simulink subsystem "M8025_Actuator"  (R2025b)
settings: Solver=VariableStepAuto  StartTime=0.0  StopTime=10.0  RelTol=1e-3
model mask{VelKp=0.00076207895, VelKi=0.0015241579}
  mask prompts: VelKp "Velocity Kp"; VelKi "Velocity Ki"
undefined symbols (not defined in the file): M8025
libraries: fl_lib x12, nesl_utility x9, slpidlib x2, ee_lib x1
settings Model: Creator=Compu  LastModifiedBy=Compu

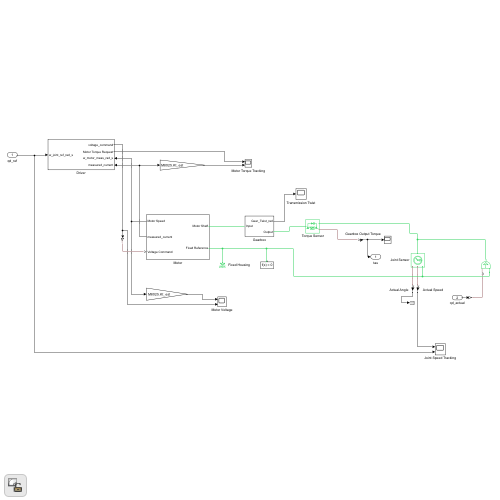
[thumbnail: Simulink's stored preview of the top-level diagram]
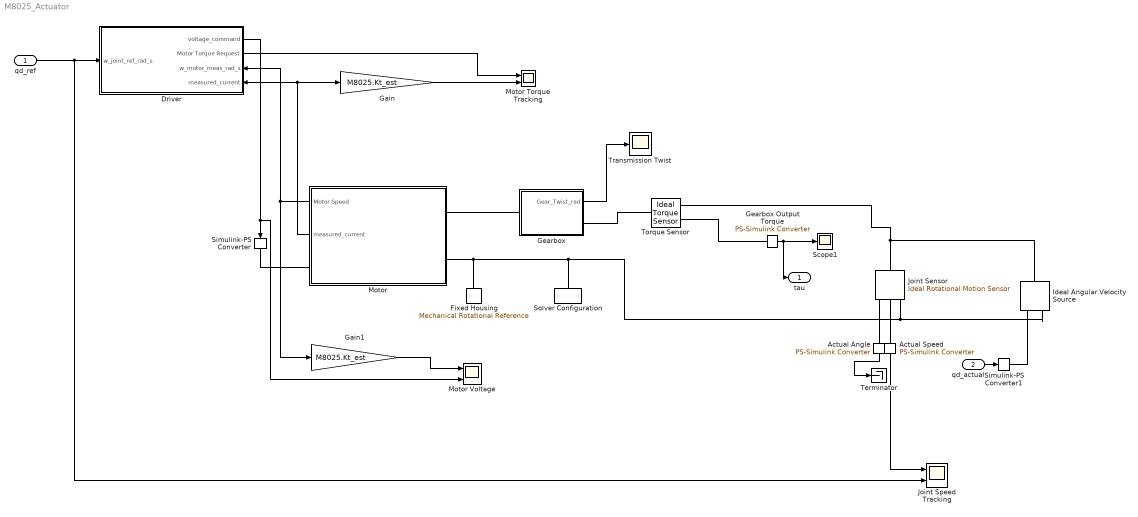
== system M8025_Actuator ==
  qd_ref : Inport
  qd_actual : Inport  Port=2
  Actual Angle : nesl_utility/PS-Simulink Converter  PhysicalDomain=network_engine_domain  SubClassName=ps_output  LeftPortType=input  RightPortType=output  PseudoPeriodic=off  Frequencies=[]  VectorFormat=inherit  Unit=rad  AffineConversion=off
  Actual Speed : nesl_utility/PS-Simulink Converter  PhysicalDomain=network_engine_domain  SubClassName=ps_output  LeftPortType=input  RightPortType=output  PseudoPeriodic=off  Frequencies=[]  VectorFormat=inherit  Unit=rad/s  AffineConversion=off
  Driver : Subsystem
      settings: PortSchema="{\"entries\":[{\"content\":{\"sides\":[{\"content\":{\"connectorIds\":[\"In1\"]},\"type\":\"ConnectorPlacement.EquallySpacedRectSide\",\"uuid\":\"4f9c6ada-d4f2-4042-b799-7a5129c92780\"},{\"content\":{\"connectorIds\":[\"Out1\",\"Out2\",\"In2\",\"In3\"],\"side\":\"RIGHT\"},\"type\":\"ConnectorPlacement.EquallySpacedRectSide\",\"uuid\":\"e7c5d0cc-560f-4bd8-9eed-f21f11202f3f\"},{\"content\":{\"side\":\"TOP\"},\"type\":\"ConnectorPlacement.EquallySpacedRectSide\",\"uuid\":\"9d50fcf4-e910-4695-a284-862e67cc701d\"}]},\"type\":\"ConnectorPlacement.EquallySpacedConnector\",\"uuid\":\"3eedfdac-378a-49e8-9696-691ddb81d7b7\"}],\"packageUris\":[\"http://schema.mathworks.com/mf0/Connector/R2020b\"],\"version\":\"1.0\"}"
  Fixed Housing : fl_lib/Mechanical/Rotational Elements/Mechanical Rotational Reference
  Gain : Gain  Gain=M8025.Kt_est
  Gain1 : Gain  Gain=M8025.Kt_est
  Gearbox : Subsystem
  Gearbox Output Torque : nesl_utility/PS-Simulink Converter  PhysicalDomain=network_engine_domain  SubClassName=ps_output  LeftPortType=input  RightPortType=output  PseudoPeriodic=off  Frequencies=[]  VectorFormat=inherit  Unit=N*m  AffineConversion=off
  Ideal Angular Velocity Source : fl_lib/Mechanical/Mechanical Sources/Ideal Angular Velocity Source
  Joint Sensor : fl_lib/Mechanical/Mechanical Sensors/Ideal Rotational Motion Sensor  reference=foundation.enum.MeasurementReference.difference  acceleration_port=false  velocity_port=true  position_port=true  wrap_angle=false  offset=0 rad
  Joint Speed Tracking : Scope  NumInputPorts=2
      settings: ActiveDisplayYMinimum=-0.02793  ActiveDisplayYMaximum=0.25141  DataLoggingVariableName=ScopeData2
  Motor : Subsystem
      settings: PortSchema="{\"entries\":[{\"content\":{\"sides\":[{\"content\":{\"connectorIds\":[\"Out1\",\"Out2\",\"LConn1\"]},\"type\":\"ConnectorPlacement.EquallySpacedRectSide\",\"uuid\":\"a7d9d3e7-63ba-44cc-8810-cbbe49fdc417\"},{\"content\":{\"connectorIds\":[\"RConn1\",\"RConn2\"],\"side\":\"RIGHT\"},\"type\":\"ConnectorPlacement.EquallySpacedRectSide\",\"uuid\":\"fa3b5d3d-db74-48e3-94ee-4f6883535878\"},{\"content\":{\"side\":\"TOP\"},\"type\":\"ConnectorPlacement.EquallySpacedRectSide\",\"uuid\":\"19ef0f19-9e47-4a9a-82bb-e035ff550378\"}]},\"type\":\"ConnectorPlacement.EquallySpacedConnector\",\"uuid\":\"8a6ad2f5-5551-4596-9ab7-1b2bcec8fe13\"}],\"packageUris\":[\"http://schema.mathworks.com/mf0/Connector/R2020b\"],\"version\":\"1.0\"}"
  Motor Torque Tracking : Scope  NumInputPorts=2
      settings: ActiveDisplayYMinimum=-0.00179  ActiveDisplayYMaximum=0.01392
  Motor Voltage : Scope  NumInputPorts=2
      settings: ActiveDisplayYMinimum=-0.49501  ActiveDisplayYMaximum=4.45509  DataLoggingVariableName=ScopeData4
  Scope1 : Scope
  Simulink-PS Converter : nesl_utility/Simulink-PS Converter  PhysicalDomain=network_engine_domain  SubClassName=ps_input  LeftPortType=input  RightPortType=output  PseudoPeriodic=off  Frequencies=[]  NoiseDistribution=none  NoiseParameters=[]  Unit=V  AffineConversion=off  FilteringAndDerivatives=provide  SimscapeFilterOrder=1  InputFilterTimeConstant=0.001  UdotUserProvided=0
  Simulink-PS Converter1 : nesl_utility/Simulink-PS Converter  PhysicalDomain=network_engine_domain  SubClassName=ps_input  LeftPortType=input  RightPortType=output  PseudoPeriodic=off  Frequencies=[]  NoiseDistribution=none  NoiseParameters=[]  Unit=1  AffineConversion=off  FilteringAndDerivatives=provide  SimscapeFilterOrder=1  InputFilterTimeConstant=0.001  UdotUserProvided=0
  Solver Configuration : nesl_utility/Solver Configuration  PhysicalDomain=network_engine_domain  SubClassName=solver  LeftPortType=input  RightPortType=generic  Tones=[]  Harmonics=[]  SimulateNoise=off  Profile=off  UseLocalSampling=off  EnableSwitchedLinearOptims=on  FrequencyDomain=off  UseCCode=off  RelTol=0.001  AbsTol=0.001  MinStep=1e-09  ToWorkspace=off  RevertToSquareIcSolve=off  NumHomotopyIterations=100  PhasorMode=off  PhasorModeNumHarmonics=1  ConsistencySolver=NEWTON_XTOL_AFTER_FTOL  IndexReductionMethod=DerivativeReplacement  DoDC=off  ResidualTolerance=1e-09  ConsistencyTolSource=GLOBAL  ConsistencyAbsTol=0.001  ConsistencyRelTol=0.001  ConsistencyTolFactor=0.001  UseLocalSolver=off  LocalSolverChoice=NE_BACKWARD_EULER_ADVANCER  ResolveIndetEquations=on  FunctionEvalNumThread=1  LocalSolverSampleTime=0.001  DoFixedCost=off  MaxNonlinIter=3  MaxModeIter=2  ComputeImpulses=off  ImpulseIterations=2  LinearAlgebra=auto  LinearAlgebraNumThread=0  EquationFormulation=NE_TIME_EF  DelaysMemoryBudget=1024  AutomaticFiltering=on  FilteringTimeConstant=0.001  PartitionStorageMethod=AS_NEEDED  PartitionMemoryBudget=1024  PartitionMethod=ROBUST  MultibodyUseLocalSolver=off  MultibodyLocalSolverChoice=ODE1  MultibodyLocalSolverSampleTime=0.001
  Terminator : Terminator
  Torque Sensor : fl_lib/Mechanical/Mechanical Sensors/Ideal Torque Sensor
  Transmission Twist : Scope
      settings: ActiveDisplayYMinimum=-2E-6  ActiveDisplayYMaximum=2E-5  DataLoggingVariableName=ScopeData5
  tau : Outport
  wires:
  Actual Speed/1 -> Joint Speed Tracking/1
  qd_actual/1 -> Simulink-PS Converter1/1
  Driver/1(voltage_command) -> Simulink-PS Converter/1, Motor Voltage/2
  qd_ref/1 -> Driver/1(w_joint_ref_rad_s), Joint Speed Tracking/2
  Motor/2(measured_current) -> Driver/3(measured_current), Gain/1
  Gearbox Output Torque/1 -> Scope1/1, tau/1
  Driver/2(Motor Torque Request) -> Motor Torque Tracking/1
  Actual Angle/1 -> Terminator/1
  Motor/1(Motor Speed) -> Driver/2(w_motor_meas_rad_s), Gain1/1
  Gain/1 -> Motor Torque Tracking/2
  Gain1/1 -> Motor Voltage/1
  Gearbox/1(Gear_Twist_rad) -> Transmission Twist/1
  connections:
  Fixed Housing/LConn1 -- Joint Sensor/RConn1 -- Ideal Angular Velocity Source/RConn2 -- Solver Configuration/RConn1 -- Motor/RConn2
  Ideal Angular Velocity Source/LConn1 -- Joint Sensor/LConn1 -- Torque Sensor/RConn1
  Torque Sensor/RConn2 -- Gearbox Output Torque/LConn1
  Simulink-PS Converter1/RConn1 -- Ideal Angular Velocity Source/RConn1
  Simulink-PS Converter/RConn1 -- Motor/LConn1
  Joint Sensor/RConn2 -- Actual Speed/LConn1
  Gearbox/RConn1 -- Torque Sensor/LConn1
  Motor/RConn1 -- Gearbox/LConn1
  Joint Sensor/RConn3 -- Actual Angle/LConn1

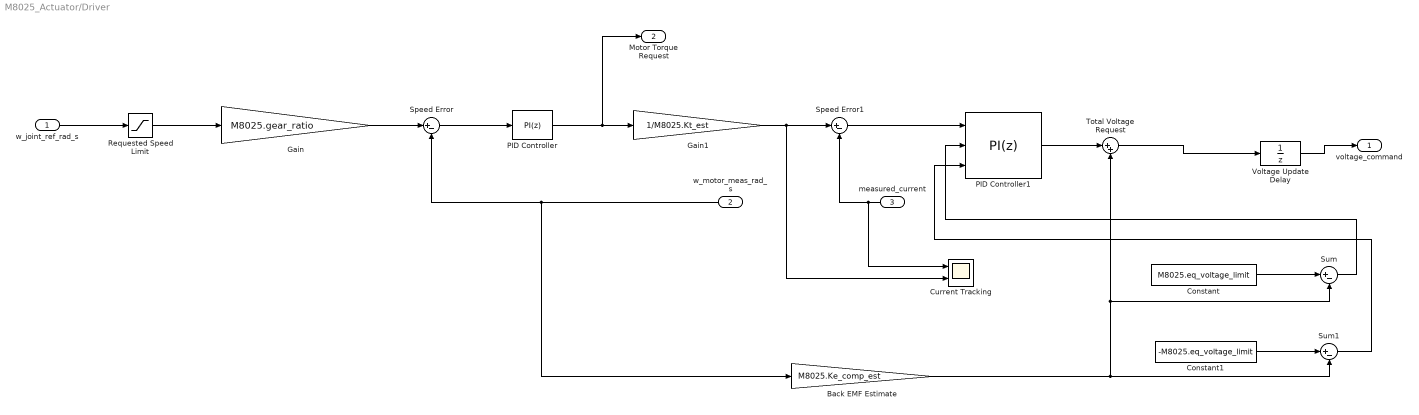
== system M8025_Actuator/Driver ==
  w_joint_ref_rad_s : Inport
  w_motor_meas_rad_s : Inport  Port=2
  measured_current : Inport  Port=3
  Back EMF Estimate : Gain  Gain=M8025.Ke_comp_est
  Constant : Constant  Value=M8025.eq_voltage_limit
  Constant1 : Constant  Value=-M8025.eq_voltage_limit
  Current Tracking : Scope  NumInputPorts=2
      settings: ActiveDisplayYMinimum=-0.00854  ActiveDisplayYMaximum=0.06628  DataLoggingVariableName=ScopeData3
  Gain : Gain  Gain=M8025.gear_ratio
  Gain1 : Gain  Gain=1/M8025.Kt_est
  PID Controller : slpidlib/PID Controller  Controller=PI  Form=Parallel  TimeDomain=Discrete-time  UseExternalTs=off  SampleTime=0.0001  IntegratorMethod=Forward Euler  FilterMethod=Forward Euler  ControllerParametersSource=internal  P=VelKp  I=VelKi  UseKiTs=off  D=0  UseExternalDerivativeSource=off  N=100  UseFilter=on  TunerSelectOption=Transfer Function Based (PID Tuner App)  InitialConditionSource=internal  InitialConditionForIntegrator=0  InitialConditionForFilter=0  DifferentiatorICPrevScaledInput=0  ExternalReset=none  TrackingMode=off  Kt=1  LimitOutput=on  SatLimitsSource=internal  UpperSaturationLimit=M8025.rated_output_torque/M8025.gear_ratio  LowerSaturationLimit=-M8025.rated_output_torque/M8025.gear_ratio  LinearizeAsGain=on  AntiWindupMode=clamping  Kb=1  LimitIntegrator=off  UpperIntegratorSaturationLimit=inf  LowerIntegratorSaturationLimit=-inf  POutMin=[]  POutMax=[]  IOutMin=[]  IOutMax=[]  DOutMin=[]  DOutMax=[]  NOutMin=[]  NOutMax=[]  SumOutMin=[]  SumOutMax=[]  SaturationOutMin=[]  SaturationOutMax=[]  PParamMin=[]  PParamMax=[]  IParamMin=[]  IParamMax=[]  DParamMin=[]  DParamMax=[]  NParamMin=[]  NParamMax=[]  KbParamMin=[]  KbParamMax=[]  KtParamMin=[]  KtParamMax=[]  KbOutMin=[]  KbOutMax=[]  KtOutMin=[]  KtOutMax=[]  IntegratorOutMin=[]  IntegratorOutMax=[]  FilterOutMin=[]  FilterOutMax=[]  SumI1OutMin=[]  SumI1OutMax=[]  SumI2OutMin=[]  SumI2OutMax=[]  SumI3OutMin=[]  SumI3OutMax=[]  SumI4OutMin=[]  SumI4OutMax=[]  SumDOutMin=[]  SumDOutMax=[]  DifferentiatorOutMin=[]  DifferentiatorOutMax=[]  FilterDiffOutCoefMin=[]  FilterDiffOutCoefMax=[]  ReciprocalOutMin=[]  ReciprocalOutMax=[]  SumDenOutMin=[]  SumDenOutMax=[]  SumNumOutMin=[]  SumNumOutMax=[]  DivideOutMin=[]  DivideOutMax=[]  UdiffTsProdOutMin=[]  UdiffTsProdOutMax=[]  NTsProdOutMin=[]  NTsProdOutMax=[]  UintegralTsProdOutMin=[]  UintegralTsProdOutMax=[]  UngainTsProdOutMin=[]  UngainTsProdOutMax=[]  ClampingZeroOutDataTypeStr=Inherit: Inherit via back propagation  ClampingZeroOutMin=[]  ClampingZeroOutMax=[]  FilterDenConstantOutDataTypeStr=Inherit: Inherit via back propagation  FilterDenConstantOutMin=[]  FilterDenConstantOutMax=[]  PCopyOutDataTypeStr=Inherit: Inherit via back propagation  PCopyOutMin=[]  PCopyOutMax=[]  NCopyOutDataTypeStr=Inherit: Inherit via back propagation  NCopyOutMin=[]  NCopyOutMax=[]  IntegratorContinuousStateAttributes=''  IntegratorStateMustResolveToSignalObject=off  IntegratorRTWStateStorageClass=Auto  FilterContinuousStateAttributes=''  FilterStateMustResolveToSignalObject=off  FilterRTWStateStorageClass=Auto  ParallelPVariant=InternalParameters  IdealPVariant=Disabled  IVariant=InternalParameters  DVariant=Disabled  IntegratorVariant=Discrete  SatVariant=Enabled  AWVariant=DiscClampingParallel  PCopyVariant=Disabled  TRVariant=Disabled  FdbkBlocksVariant=Forward  IdealPFdbkVariant=Disabled  SatFdbkVariant=Disabled  DerivativeFilterVariant=Disabled  NVariant=Disabled  NCopyVariant=Disabled_SignalSpec  FilterICVariant=Disabled  IntegratorICVariant=InternalICs  ExternalResetVariant=Disabled  TRSumVariant=Passthrough  SumFdbkVariant=Disabled  SumVariant=Sum_PI  TsampFilterVariant=InternalTs  TsampNgainVariant=Passthrough  TsampIntegralVariant=Disabled_SignalSpec  ExternalSaturationOutDataTypeStr=Inherit: Same as second input  DerivativeSourceVariant=Disabled  PreIntVariant=InternalPreInt
  PID Controller1 : slpidlib/PID Controller  Controller=PI  Form=Parallel  TimeDomain=Discrete-time  UseExternalTs=off  SampleTime=0.0001  IntegratorMethod=Forward Euler  FilterMethod=Forward Euler  ControllerParametersSource=internal  P=M8025.current_P_design  I=M8025.current_I_design  UseKiTs=off  D=0  UseExternalDerivativeSource=off  N=100  UseFilter=on  TunerSelectOption=Transfer Function Based (PID Tuner App)  InitialConditionSource=internal  InitialConditionForIntegrator=0  InitialConditionForFilter=0  DifferentiatorICPrevScaledInput=0  ExternalReset=none  TrackingMode=off  Kt=1  LimitOutput=on  SatLimitsSource=external  UpperSaturationLimit=M8025.eq_voltage_limit  LowerSaturationLimit=-M8025.eq_voltage_limit  LinearizeAsGain=on  AntiWindupMode=clamping  Kb=1  LimitIntegrator=off  UpperIntegratorSaturationLimit=inf  LowerIntegratorSaturationLimit=-inf  POutMin=[]  POutMax=[]  IOutMin=[]  IOutMax=[]  DOutMin=[]  DOutMax=[]  NOutMin=[]  NOutMax=[]  SumOutMin=[]  SumOutMax=[]  SaturationOutMin=[]  SaturationOutMax=[]  PParamMin=[]  PParamMax=[]  IParamMin=[]  IParamMax=[]  DParamMin=[]  DParamMax=[]  NParamMin=[]  NParamMax=[]  KbParamMin=[]  KbParamMax=[]  KtParamMin=[]  KtParamMax=[]  KbOutMin=[]  KbOutMax=[]  KtOutMin=[]  KtOutMax=[]  IntegratorOutMin=[]  IntegratorOutMax=[]  FilterOutMin=[]  FilterOutMax=[]  SumI1OutMin=[]  SumI1OutMax=[]  SumI2OutMin=[]  SumI2OutMax=[]  SumI3OutMin=[]  SumI3OutMax=[]  SumI4OutMin=[]  SumI4OutMax=[]  SumDOutMin=[]  SumDOutMax=[]  DifferentiatorOutMin=[]  DifferentiatorOutMax=[]  FilterDiffOutCoefMin=[]  FilterDiffOutCoefMax=[]  ReciprocalOutMin=[]  ReciprocalOutMax=[]  SumDenOutMin=[]  SumDenOutMax=[]  SumNumOutMin=[]  SumNumOutMax=[]  DivideOutMin=[]  DivideOutMax=[]  UdiffTsProdOutMin=[]  UdiffTsProdOutMax=[]  NTsProdOutMin=[]  NTsProdOutMax=[]  UintegralTsProdOutMin=[]  UintegralTsProdOutMax=[]  UngainTsProdOutMin=[]  UngainTsProdOutMax=[]  ClampingZeroOutDataTypeStr=Inherit: Inherit via back propagation  ClampingZeroOutMin=[]  ClampingZeroOutMax=[]  FilterDenConstantOutDataTypeStr=Inherit: Inherit via back propagation  FilterDenConstantOutMin=[]  FilterDenConstantOutMax=[]  PCopyOutDataTypeStr=Inherit: Inherit via back propagation  PCopyOutMin=[]  PCopyOutMax=[]  NCopyOutDataTypeStr=Inherit: Inherit via back propagation  NCopyOutMin=[]  NCopyOutMax=[]  IntegratorContinuousStateAttributes=''  IntegratorStateMustResolveToSignalObject=off  IntegratorRTWStateStorageClass=Auto  FilterContinuousStateAttributes=''  FilterStateMustResolveToSignalObject=off  FilterRTWStateStorageClass=Auto  ParallelPVariant=InternalParameters  IdealPVariant=Disabled  IVariant=InternalParameters  DVariant=Disabled  IntegratorVariant=Discrete  SatVariant=External  AWVariant=DiscClampingParallel  PCopyVariant=Disabled  TRVariant=Disabled  FdbkBlocksVariant=Forward  IdealPFdbkVariant=Disabled  SatFdbkVariant=Disabled  DerivativeFilterVariant=Disabled  NVariant=Disabled  NCopyVariant=Disabled_SignalSpec  FilterICVariant=Disabled  IntegratorICVariant=InternalICs  ExternalResetVariant=Disabled  TRSumVariant=Passthrough  SumFdbkVariant=Disabled  SumVariant=Sum_PI  TsampFilterVariant=InternalTs  TsampNgainVariant=Passthrough  TsampIntegralVariant=Disabled_SignalSpec  ExternalSaturationOutDataTypeStr=Inherit: Same as second input  DerivativeSourceVariant=Disabled  PreIntVariant=InternalPreInt
  Requested Speed Limit : Saturate  UpperLimit=1.885  LowerLimit=-1.885
  Speed Error : Sum  Inputs=|+-
  Speed Error1 : Sum  Inputs=|+-
  Sum : Sum  Inputs=|+-
  Sum1 : Sum  Inputs=|+-
  Total Voltage Request : Sum  Inputs=|++
  Voltage Update Delay : UnitDelay  SampleTime=0.0001  HasFrameUpgradeWarning=on
  voltage_command : Outport
  Motor Torque Request : Outport  Port=2
  wires:
  Constant1/1 -> Sum1/1
  Sum1/1 -> PID Controller1/3
  Sum/1 -> PID Controller1/2
  Constant/1 -> Sum/1
  PID Controller1/1 -> Total Voltage Request/1
  Back EMF Estimate/1 -> Sum/2, Total Voltage Request/2, Sum1/2
  measured_current/1 -> Speed Error1/2, Current Tracking/1
  Speed Error1/1 -> PID Controller1/1
  Gain1/1 -> Speed Error1/1, Current Tracking/2
  PID Controller/1 -> Gain1/1, Motor Torque Request/1
  w_joint_ref_rad_s/1 -> Requested Speed Limit/1
  Gain/1 -> Speed Error/1
  Speed Error/1 -> PID Controller/1
  Requested Speed Limit/1 -> Gain/1
  w_motor_meas_rad_s/1 -> Back EMF Estimate/1, Speed Error/2
  Total Voltage Request/1 -> Voltage Update Delay/1
  Voltage Update Delay/1 -> voltage_command/1

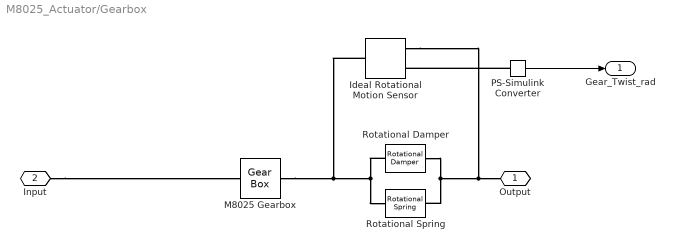
== system M8025_Actuator/Gearbox ==
  Ideal Rotational Motion Sensor : fl_lib/Mechanical/Mechanical Sensors/Ideal Rotational Motion Sensor  reference=foundation.enum.MeasurementReference.difference  acceleration_port=false  velocity_port=false  position_port=true  wrap_angle=false  offset=0 rad
      settings: InternalSimscapePortConfiguration="{\"Bottom\":[],\"Left\":[{\"id\":\"R\",\"label\":\"R\",\"type\":\"foundation.mechanical.rotational.rotational\"}],\"Right\":[{\"id\":\"C\",\"label\":\"C\",\"type\":\"foundation.mechanical.rotational.rotational\"},{\"id\":\"A\",\"label\":\"A\",\"type\":\"output\"}],\"Top\":[]}"
  M8025 Gearbox : fl_lib/Mechanical/Mechanisms/Gear Box  ratio=M8025.gear_ratio  t_in_specify=off  t_in_priority=None  t_in=0 N*m  t_in_nominal_specify=off  t_in_nominal_value=1  t_in_nominal_unit=N*m  t_out_specify=off  t_out_priority=None  t_out=0 N*m  t_out_nominal_specify=off  t_out_nominal_value=1  t_out_nominal_unit=N*m
  PS-Simulink Converter : nesl_utility/PS-Simulink Converter  PhysicalDomain=network_engine_domain  SubClassName=ps_output  LeftPortType=input  RightPortType=output  PseudoPeriodic=off  Frequencies=[]  VectorFormat=inherit  Unit=rad  AffineConversion=off
  Rotational Damper : fl_lib/Mechanical/Rotational Elements/Rotational Damper  D=M8025.gear_damping_trial N*m*s/rad  w_specify=off  w_priority=None  w=0 rad/s  w_nominal_specify=off  w_nominal_value=1  w_nominal_unit=rad/s  t_specify=off  t_priority=None  t=0 N*m  t_nominal_specify=off  t_nominal_value=1  t_nominal_unit=N*m
  Rotational Spring : fl_lib/Mechanical/Rotational Elements/Rotational Spring  spr_rate=M8025.gear_stiffness_trial N*m/rad  w_specify=off  w_priority=None  w=0 rad/s  w_nominal_specify=off  w_nominal_value=1  w_nominal_unit=rad/s  t_specify=off  t_priority=None  t=0 N*m  t_nominal_specify=off  t_nominal_value=1  t_nominal_unit=N*m  phi_specify=off  phi_priority=High  phi=0 rad  phi_nominal_specify=off  phi_nominal_value=1  phi_nominal_unit=rad
  Output : PMIOPort  Side=Right
  Input : PMIOPort  Port=2  Side=Left
  Gear_Twist_rad : Outport
  wires:
  PS-Simulink Converter/1 -> Gear_Twist_rad/1
  connections:
  PS-Simulink Converter/LConn1 -- Ideal Rotational Motion Sensor/RConn2
  Rotational Spring/RConn1 -- Output/RConn1 -- Ideal Rotational Motion Sensor/RConn1 -- Rotational Damper/RConn1
  Rotational Spring/LConn1 -- M8025 Gearbox/RConn1 -- Ideal Rotational Motion Sensor/LConn1 -- Rotational Damper/LConn1
  Input/RConn1 -- M8025 Gearbox/LConn1

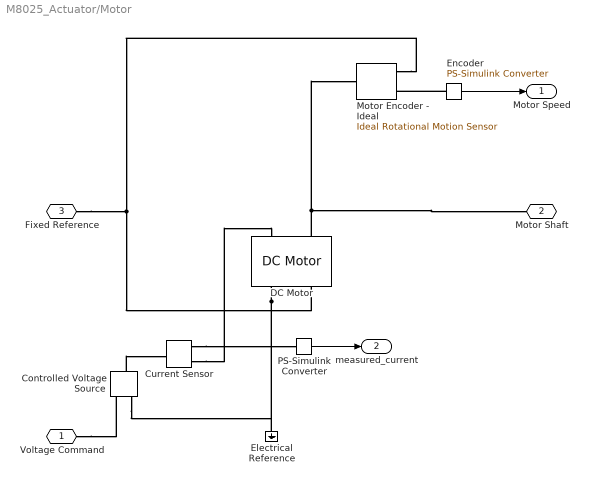
== system M8025_Actuator/Motor ==
  Controlled Voltage Source : fl_lib/Electrical/Electrical Sources/Controlled Voltage Source
  Current Sensor : fl_lib/Electrical/Electrical Sensors/Current Sensor
  DC Motor : ee_lib/Electromechanical/Brushed Motors/DC Motor  field_option=ee.enum.field_option.pm  Rf=100 Ohm  Lf=1 H  Laf=0.15 H  If0=0 A  parameterization=ee.enum.dcparam_option.circuit_param  Ra=M8025.eq_R Ohm  La=M8025.eq_L H  emf_or_torque=ee.enum.emf_or_torque.ki  Kv=0.072e-3 V/rpm  Ki=M8025.Kt_est N*m/A  T_stall=0.24e-3 N*m  w_max=19100 rpm  w_rated=15000 rpm  P_rated=0.08 W  V_rated=1.5 V  lam_param=ee.enum.lam_param.damping  i_noload=0 A  V_i_noload=1.5 V  J=M8025.rotor_inertia kg*m^2  lam=0 N*m*s/rad  speed0=0 rpm  alpha=3.93e-3 1/K  Tmeas=25 degC  thermal_mass=100 J/K  initial_temperature=25 degC
  Electrical Reference : fl_lib/Electrical/Electrical Elements/Electrical Reference
  Encoder : nesl_utility/PS-Simulink Converter  PhysicalDomain=network_engine_domain  SubClassName=ps_output  LeftPortType=input  RightPortType=output  PseudoPeriodic=off  Frequencies=[]  VectorFormat=inherit  Unit=rad/s  AffineConversion=off
  Motor Encoder - Ideal : fl_lib/Mechanical/Mechanical Sensors/Ideal Rotational Motion Sensor  reference=foundation.enum.MeasurementReference.difference  acceleration_port=false  velocity_port=true  position_port=false  wrap_angle=false  offset=0 rad
      settings: InternalSimscapePortConfiguration="{\"Bottom\":[],\"Left\":[{\"id\":\"R\",\"label\":\"R\",\"type\":\"foundation.mechanical.rotational.rotational\"}],\"Right\":[{\"id\":\"C\",\"label\":\"C\",\"type\":\"foundation.mechanical.rotational.rotational\"},{\"id\":\"W\",\"label\":\"W\",\"type\":\"output\"}],\"Top\":[]}"
  PS-Simulink Converter : nesl_utility/PS-Simulink Converter  PhysicalDomain=network_engine_domain  SubClassName=ps_output  LeftPortType=input  RightPortType=output  PseudoPeriodic=off  Frequencies=[]  VectorFormat=inherit  Unit=A  AffineConversion=off
  Voltage Command : PMIOPort  Side=Left
  Motor Shaft : PMIOPort  Port=2  Side=Right
  Fixed Reference : PMIOPort  Port=3  Side=Right
  Motor Speed : Outport
  measured_current : Outport  Port=2
  wires:
  PS-Simulink Converter/1 -> measured_current/1
  Encoder/1 -> Motor Speed/1
  connections:
  Current Sensor/RConn1 -- PS-Simulink Converter/LConn1
  DC Motor/RConn1 -- Electrical Reference/LConn1 -- Controlled Voltage Source/RConn2
  Current Sensor/RConn2 -- DC Motor/LConn1
  Controlled Voltage Source/LConn1 -- Current Sensor/LConn1
  Motor Encoder - Ideal/RConn1 -- DC Motor/RConn2 -- Fixed Reference/RConn1
  Encoder/LConn1 -- Motor Encoder - Ideal/RConn2
  DC Motor/LConn2 -- Motor Encoder - Ideal/LConn1 -- Motor Shaft/RConn1
  Voltage Command/RConn1 -- Controlled Voltage Source/RConn1
